simulink model "Fault_Line_2018"  (R2018b)
settings: Solver=VariableStepAuto  StartTime=0.0  StopTime=0.2  FixedStep=1/12000  RelTol=1e-3
undefined symbols (not defined in the file or in its folder): D1, D11, Delta
libraries: powerlib x16, spsGroundingTransformerLib x1
settings Model: SimulationMode=accelerator  Creator=zyx  LastModifiedBy=zyx53
settings DebuggingCC: UnconnectedInputMsg=none  UnconnectedOutputMsg=none  UnconnectedLineMsg=none
settings ModelReferenceCC: EnableRefExpFcnMdlSchedulingChecks=off
settings RTWCC: Description=Generic Real-Time Target

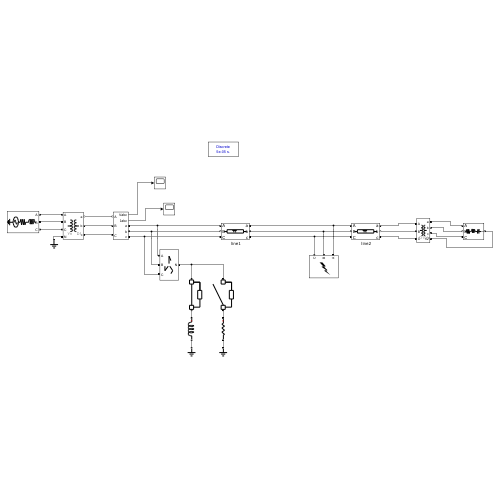
[thumbnail: Simulink's stored preview of the top-level diagram]
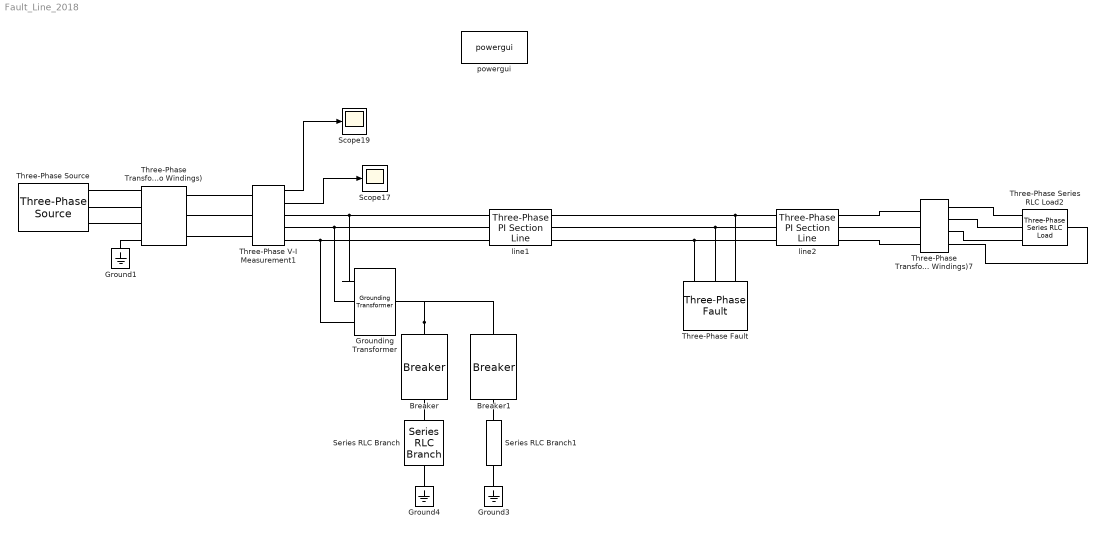
== system Fault_Line_2018 ==
  " line1" : powerlib/Elements/Three-Phase PI Section Line  LConnTagsString=a|b|c  RConnTagsString=A|B|C  Length=9  Frequency=50  Resistances=[0.17 0.23]  Inductances="[1.21e-3  5.48e-3]"  Capacitances="[9.7e-9  6e-9]"
  " line2" : powerlib/Elements/Three-Phase PI Section Line  LConnTagsString=a|b|c  RConnTagsString=A|B|C  Length=1  Frequency=50  Resistances=[0.17 0.23]  Inductances="[1.21e-3  5.48e-3]"  Capacitances="[9.7e-9  6e-9]"
  Breaker : powerlib/Elements/Breaker  InitialState=1  SwitchingTimes=5  External=off  BreakerResistance=0.01  SnubberResistance=1e6  SnubberCapacitance=inf  Measurements=None  MoreParameters=on  NoBreakLoop=off
  Breaker1 : powerlib/Elements/Breaker  InitialState=0  SwitchingTimes=5  External=off  BreakerResistance=0.01  SnubberResistance=1e6  SnubberCapacitance=inf  Measurements=None  MoreParameters=on  NoBreakLoop=off
  Ground1 : powerlib/Elements/Ground  LConnTagsString=a
  Ground3 : powerlib/Elements/Ground  LConnTagsString=a
  Ground4 : powerlib/Elements/Ground  LConnTagsString=a
  "Grounding Transformer " : spsGroundingTransformerLib/Grounding Transformer   UNITS=pu  NominalPower="[100e6   50]"  NominalVoltage=10e3  ZeroSequenceImpedance_pu=[0.025 0.75]  MagnetizationBranch_pu=[500 500]  ZeroSequenceImpedance_SI=[0.052083 589.05]  MagnetizationBranch_SI=[1041.7 3.927e+005]  Measurements=None
  Scope17 : Scope
  Scope19 : Scope
  Series RLC Branch : powerlib/Elements/Series RLC Branch  LConnTagsString=__new0  RConnTagsString=__new0  BranchType=L  Resistance=1  Inductance=0.1  SetiL0=off  InitialCurrent=0  Capacitance=1e-6  Setx0=off  InitialVoltage=0  Measurements=None
  Series RLC Branch1 : powerlib/Elements/Series RLC Branch  LConnTagsString=__new0  RConnTagsString=__new0  BranchType=R  Resistance=40  Inductance=1e-3  SetiL0=off  InitialCurrent=0  Capacitance=1e-6  Setx0=off  InitialVoltage=0  Measurements=None
  Three-Phase Series RLC Load2 : powerlib/Elements/Three-Phase Series RLC Load  LConnTagsString=A|B|C  RConnTagsString=N  Configuration=Y (neutral)  NominalVoltage=380  Vabc=[1e3 1e3 1e3]  Vabcp=[1e3 1e3 1e3]  NominalFrequency=50  UnbalancedPower=off  ActivePower=360e3  InductivePower=194e3  CapacitivePower=75e3  Pabc=[10e3 9e3 11e3]  QLabc=[100 90 110]  QCabc=[100 90 110]  Pabcp=[10e3 9e3 11e3]  QLabcp=[100 90 110]  QCabcp=[100 90 110]  Measurements=None  LoadType=constant Z
  Three-Phase Transformer (Two Windings) : powerlib/Elements/Three-Phase Transformer (Two Windings)  Winding1Connection=Yn  Winding2Connection=Delta (D1)  CoreType=Three single-phase transformers  SetSaturation=off  Hysteresis=off  DataFile='hysteresis'  SetInitialFlux=off  Measurements=None  UNITS=pu  NominalPower=[ 4000e3 , 50 ]  Winding1=[ 110e3 , 0.002 , 0.08 ]  Winding2=[ 10e3 , 0.002 , 0.08 ]  Rm=1000  Lm=500  L0=0.5  Saturation=[ 0,0 ; 0.0024,1.2 ; 1.0,1.52 ]  InitialFluxes=[ 0.8 , -0.8 , 0.7 ]  BreakLoop=off  DiscreteSolver=Trapezoidal iterative  DataType=off  TransfoNumber=1
  Three-Phase Transformer (Two Windings)7 : powerlib/Elements/Three-Phase Transformer (Two Windings)  Winding1Connection=Delta (D11)  Winding2Connection=Yn  CoreType=Three single-phase transformers  SetSaturation=off  Hysteresis=off  DataFile='hysteresis'  SetInitialFlux=off  Measurements=None  UNITS=pu  NominalPower=[ 400e3 , 50 ]  Winding1=[ 10e3 , 0.002 , 0.08 ]  Winding2=[ 0.4e3 , 0.002 , 0.08 ]  Rm=500  Lm=500  L0=0.5  Saturation=[ 0,0 ; 0.0024,1.2 ; 1.0,1.52 ]  InitialFluxes=[ 0.8 , -0.8 , 0.7 ]  BreakLoop=off  DiscreteSolver=Trapezoidal iterative  DataType=off  TransfoNumber=1
  Three-Phase V-I Measurement1 : powerlib/Measurements/Three-Phase V-I Measurement  VoltageMeasurement=phase-to-phase  SetLabelV=off  LabelV=U4  Vpu=off  VpuLL=off  CurrentMeasurement=yes  SetLabelI=off  LabelI=I4  Ipu=off  Pbase=100e6  Vbase=500e3  OutputType=Complex  PhasorSimulation=off  PSBequivalent=0
  Three-Phase Fault : powerlib/Elements/Three-Phase Fault  InitialStates=0  FaultA=on  FaultB=on  FaultC=on  GroundFault=off  SwitchTimes="[0.065  0.1]"  External=off  SwitchStatus=NaN  FaultResistance=0.001  GroundResistance=0.01  SnubberResistance=1e6  SnubberCapacitance=inf  Measurements=None
  Three-Phase Source : powerlib/Electrical Sources/Three-Phase Source  InternalConnection=Yg  VoltagePhases=off  Voltage=110e3  PhaseAngle=0  Voltage_phases=[25e3 25e3 25e3]/sqrt(3)  PhaseAngles_phases=[0 -120 +120]  Frequency=50  NonIdealSource=on  SpecifyImpedance=off  Resistance=0.8929  Inductance=16.58e-3  ShortCircuitLevel=30e6  BaseVoltage=110e3  XRratio=7  BusType=swing  Pref=10e3  Qref=0  Prefabc=[10e3, 10e3, 10e3]  Qrefabc=[0, 0, 0]  Qmin=-inf  Qmax=inf
  powergui : powerlib/powergui  Priority=1  SimulationMode=Discrete  SampleTime=50e-6  frequency=60  Iterations=50  frequencyindice=50  Pbase=100e6  ErrMax=1e-4  UnitsV=kV  UnitsW=MW  buscounter=0  FunctionMessages=off  echomessages=off  EnableUseOfTLC=off  CurrentSourceSwitches=off  DisableSnubberDevices=off  DisableRonSwitches=off  DisableVfSwitches=off  DisplayEquations=off  AutomaticDiscreteSolvers=off  SolverType=Tustin/Backward Euler (TBE)  Interpol=off  ExternalGateDelay=off  methode=off  Ts=100  x0status=blocks  SPID=on  SwTol=0  HookPort=off  NonlinearTolerance=1e-4  nMaxIteration=100  ContinueOnMaxIteration=off  RestoreLinks=warning  ResistiveCurrentMeasurement=off  Frange=[0:2:500]  Ylog=off  Xlog=on  ShowGrid=off  save=off  variable=ZData  structure=0  ZoomFFT=off  StartTime=0.0  cycles=1  DisplayStyle=1  fundamental=60  FreqAxis=off  MaxFrequency=1000  frequencyindicesteady=1  RmsSteady=1  display=off
  wires:
  Three-Phase V-I Measurement1/1 -> Scope19/1
  Three-Phase V-I Measurement1/2 -> Scope17/1
  connections:
  " line1"/RConn1 -- " line2"/LConn1 -- Three-Phase Fault/LConn1
  " line1"/RConn2 -- " line2"/LConn2 -- Three-Phase Fault/LConn2
  " line1"/RConn3 -- " line2"/LConn3 -- Three-Phase Fault/LConn3
  Three-Phase V-I Measurement1/RConn1 -- " line1"/LConn1 -- "Grounding Transformer "/LConn1
  Breaker/RConn1 -- "Grounding Transformer "/RConn1 -- Breaker1/RConn1
  Three-Phase V-I Measurement1/RConn2 -- " line1"/LConn2 -- "Grounding Transformer "/LConn2
  Three-Phase V-I Measurement1/RConn3 -- " line1"/LConn3 -- "Grounding Transformer "/LConn3
  Ground3/LConn1 -- Series RLC Branch1/RConn1
  Three-Phase Transformer (Two Windings)/RConn2 -- Three-Phase V-I Measurement1/LConn2
  Three-Phase Transformer (Two Windings)/RConn1 -- Three-Phase V-I Measurement1/LConn1
  Three-Phase Transformer (Two Windings)/RConn3 -- Three-Phase V-I Measurement1/LConn3
  Ground4/LConn1 -- Series RLC Branch/RConn1
  Breaker1/LConn1 -- Series RLC Branch1/LConn1
  Series RLC Branch/LConn1 -- Breaker/LConn1
  Three-Phase Transformer (Two Windings)7/LConn2 -- " line2"/RConn2
  " line2"/RConn1 -- Three-Phase Transformer (Two Windings)7/LConn1
  Three-Phase Transformer (Two Windings)7/RConn1 -- Three-Phase Series RLC Load2/LConn1
  " line2"/RConn3 -- Three-Phase Transformer (Two Windings)7/LConn3
  Three-Phase Transformer (Two Windings)7/RConn2 -- Three-Phase Series RLC Load2/LConn2
  Three-Phase Transformer (Two Windings)7/RConn3 -- Three-Phase Series RLC Load2/LConn3
  Three-Phase Series RLC Load2/RConn1 -- Three-Phase Transformer (Two Windings)7/RConn4
  Three-Phase Transformer (Two Windings)/LConn4 -- Ground1/LConn1
  Three-Phase Source/RConn1 -- Three-Phase Transformer (Two Windings)/LConn1
  Three-Phase Source/RConn3 -- Three-Phase Transformer (Two Windings)/LConn3
  Three-Phase Source/RConn2 -- Three-Phase Transformer (Two Windings)/LConn2
